simulink model "adc_behavioral"  (R2026a)
settings: Solver=FixedStepDiscrete  StartTime=0  StopTime=4095  FixedStep=1
model workspace (MAT data in the model file):
  C.digital_mode = 3
  C.initial1 = [1 1 1 1]
  C.initial2 = [1 1 1 1]
  C.initial_analog = [0 0 0]
  C.mu1 = [3.81469726563e-09 1.14440917969e-08 2.28881835938e-08 4.57763671875e-08]
  C.mu2 = [6.103515625e-08 1.8310546875e-07 3.662109375e-07 7.32421875e-07]
  C.aux1_gain = 1
  C.aux1_offset = 0
  C.dither_amplitude = 0.03125
  C.copy1 = 64
  C.copy2 = 16
  C.s1_thresholds = [-0.875 -0.625 -0.375 -0.125 0.125 0.375 0.625 0.875]
  C.s1_levels = [-1 -0.75 -0.5 -0.25 0 0.25 0.5 0.75 1]
  C.s1_errors = [0 0 0 0 0 0 0 0 0]
  C.s1_gain = 4
  C.s1_analog = [1 0.975 -0.055 1 0 0.25 0.5 0.75 1 0 0.25 0.5 0.75 1]
  C.s1_phase = [0 0.04 1 0]
  C.s2_thresholds = [-0.875 -0.625 -0.375 -0.125 0.125 0.375 0.625 0.875]
  C.s2_levels = [-1 -0.75 -0.5 -0.25 0 0.25 0.5 0.75 1]
  C.s2_errors = [0 0 0 0 0 0 0 0 0]
  C.s2_gain = 4
  C.s2_analog = [1 0.98 -0.04 1 0 0.25 0.5 0.75 1 0 0.25 0.5 0.75 1]
  C.s2_phase = [0 0.03 1 0]
  C.aux_parameters = [0 1 0 4 4 1 0 1 0.06 1 0]
  d1_signal = [0 1 2 3 4 5 6 7 8 9 10 11 ... (8192 elements, 4096x2)]
  d2_signal = [0 1 2 3 4 5 6 7 8 9 10 11 ... (8192 elements, 4096x2)]
  n_signal = [0 1 2 3 4 5 6 7 8 9 10 11 ... (8192 elements, 4096x2)]
  x_signal = [0 1 2 3 4 5 6 7 8 9 10 11 ... (8192 elements, 4096x2)]
values from neighbouring files (symbols this model uses):
  C = entry.parameters    [adc_load_case.m]    (also in audit_adc_model.m = evalin(workspace,'C'))
(part 1 of 2)
Description:
  | Gu behavioral ADC: independent Simulink implementation, one tick per conversion.
settings Model: Creator=17765  LastModifiedBy=17765

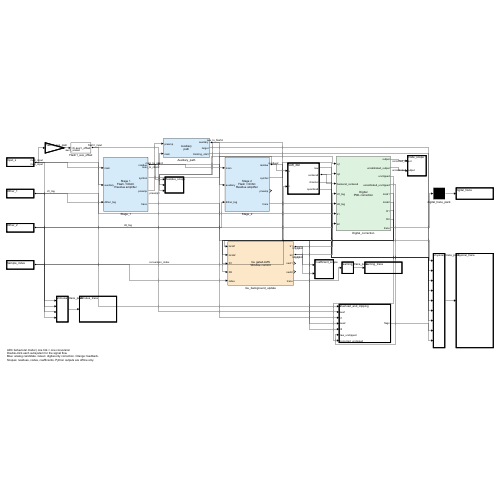
[thumbnail: Simulink's stored preview of the top-level diagram]
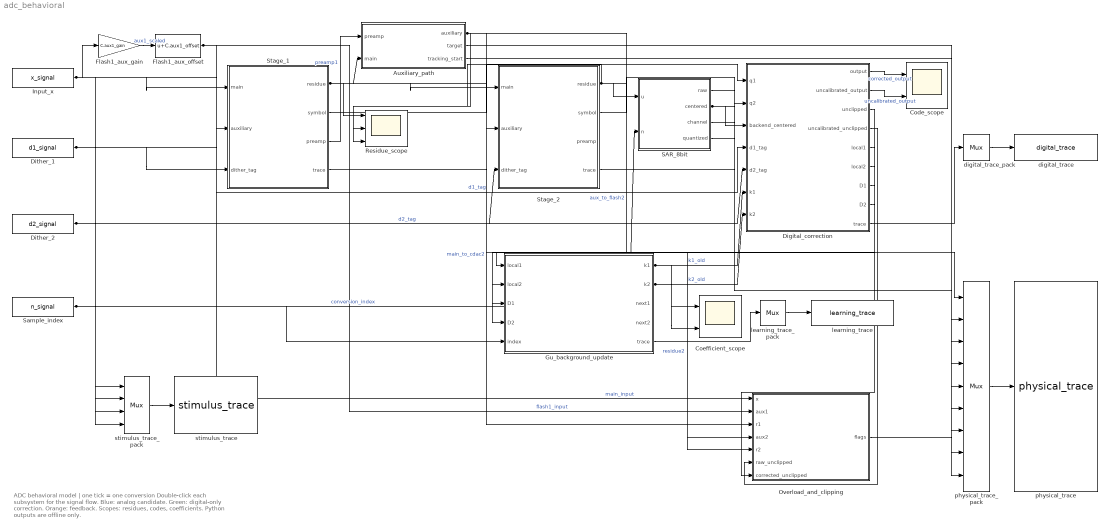
== system adc_behavioral ==
  note: ADC behavioral model | one tick = one conversion
      | Double-click each subsystem for the signal flow.
      | Blue: analog candidate. Green: digital-only correction. Orange: feedback.
      | Scopes: residues, codes, coefficients. Python outputs are offline only.
  Auxiliary_path : Subsystem
      settings: OpenFcn=open_system(gcb,'force')
      mask Display: disp(sprintf('Auxiliary\npath'));
  Code_scope : Scope  NumInputPorts=2
  Coefficient_scope : Scope  NumInputPorts=2
  Digital_correction : Subsystem
      settings: OpenFcn=open_system(gcb,'force')
      mask Display: disp(sprintf('Digital\nPWL correction'));
  Dither_1 : FromWorkspace  VariableName=d1_signal  SampleTime=1  Interpolate=off  OutputAfterFinalValue=Holding final value
  Dither_2 : FromWorkspace  VariableName=d2_signal  SampleTime=1  Interpolate=off  OutputAfterFinalValue=Holding final value
  Flash1_aux_gain : Gain  Gain=C.aux1_gain
  Flash1_aux_offset : Bias  Bias=C.aux1_offset  SaturateOnIntegerOverflow=off
  Gu_background_update : Subsystem
      settings: OpenFcn=open_system(gcb,'force')
      mask Display: disp(sprintf('Gu gated-LMS\nWindow commit'));
  Input_x : FromWorkspace  VariableName=x_signal  SampleTime=1  Interpolate=off  OutputAfterFinalValue=Holding final value
  Overload_and_clipping : MATLAB Function  TreatAsAtomicUnit=on
  Residue_scope : Scope  NumInputPorts=3
  SAR_8bit : MATLAB Function  TreatAsAtomicUnit=on
  Sample_index : FromWorkspace  VariableName=n_signal  SampleTime=1  Interpolate=off  OutputAfterFinalValue=Holding final value
  Stage_1 : Subsystem
      settings: OpenFcn=open_system(gcb,'force')
      mask Display: disp(sprintf('Stage 1\nFlash / CDAC\nResidue amplifier'));
  Stage_2 : Subsystem
      settings: OpenFcn=open_system(gcb,'force')
      mask Display: disp(sprintf('Stage 2\nFlash / CDAC\nResidue amplifier'));
  digital_trace : ToWorkspace  VariableName=digital_trace  SampleTime=1
  digital_trace_pack : Mux  Inputs=1
  learning_trace : ToWorkspace  VariableName=learning_trace  SampleTime=1
  learning_trace_pack : Mux  Inputs=1
  physical_trace : ToWorkspace  VariableName=physical_trace  SampleTime=1
  physical_trace_pack : Mux  Inputs=9
  stimulus_trace : ToWorkspace  VariableName=stimulus_trace  SampleTime=1
  stimulus_trace_pack : Mux
  wires:
  Input_x/1 -> Flash1_aux_gain/1, Stage_1/1(main), Overload_and_clipping/1(x), stimulus_trace_pack/2  "main_input"
  Flash1_aux_gain/1 -> Flash1_aux_offset/1  "aux1_scaled"
  Flash1_aux_offset/1 -> Stage_1/2(auxiliary), Overload_and_clipping/2(aux1)  "flash1_input"
  Dither_1/1 -> Stage_1/3(dither_tag), Digital_correction/4(d1_tag), stimulus_trace_pack/3  "d1_tag"
  Stage_1/3(preamp) -> Auxiliary_path/1(preamp)  "preamp1"
  Stage_1/1(residue) -> Auxiliary_path/2(main), Stage_2/1(main), Residue_scope/1, Overload_and_clipping/3(r1)  "main_to_cdac2"
  Auxiliary_path/1(auxiliary) -> Stage_2/2(auxiliary), Residue_scope/2, Overload_and_clipping/4(aux2)  "aux_to_flash2"
  Dither_2/1 -> Stage_2/3(dither_tag), Digital_correction/5(d2_tag), stimulus_trace_pack/4  "d2_tag"
  Stage_2/1(residue) -> SAR_8bit/1(u), Residue_scope/3, Overload_and_clipping/5(r2)  "residue2"
  Sample_index/1 -> SAR_8bit/2(n), Gu_background_update/5(index), stimulus_trace_pack/1  "conversion_index"
  Stage_1/2(symbol) -> Digital_correction/1(q1)
  Stage_2/2(symbol) -> Digital_correction/2(q2)
  SAR_8bit/2(centered) -> Digital_correction/3(backend_centered), physical_trace_pack/6
  Gu_background_update/1(k1) -> Digital_correction/6(k1), Coefficient_scope/1  "k1_old"
  Gu_background_update/2(k2) -> Digital_correction/7(k2), Coefficient_scope/2  "k2_old"
  Digital_correction/5(local1) -> Gu_background_update/1(local1)
  Digital_correction/6(local2) -> Gu_background_update/2(local2)
  Digital_correction/7(D1) -> Gu_background_update/3(D1)
  Digital_correction/8(D2) -> Gu_background_update/4(D2)
  Digital_correction/1(output) -> Code_scope/1  "corrected_output"
  Digital_correction/2(uncalibrated_output) -> Code_scope/2  "uncalibrated_output"
  Digital_correction/4(uncalibrated_unclipped) -> Overload_and_clipping/6(raw_unclipped)
  Digital_correction/3(unclipped) -> Overload_and_clipping/7(corrected_unclipped)
  Stage_1/4(trace) -> physical_trace_pack/1
  Stage_2/4(trace) -> physical_trace_pack/2
  Auxiliary_path/2(target) -> physical_trace_pack/3
  Auxiliary_path/3(tracking_start) -> physical_trace_pack/4
  SAR_8bit/1(raw) -> physical_trace_pack/5
  SAR_8bit/3(channel) -> physical_trace_pack/7
  SAR_8bit/4(quantized) -> physical_trace_pack/8
  Overload_and_clipping/1(flags) -> physical_trace_pack/9
  physical_trace_pack/1 -> physical_trace/1
  Digital_correction/9(trace) -> digital_trace_pack/1
  digital_trace_pack/1 -> digital_trace/1
  Gu_background_update/5(trace) -> learning_trace_pack/1
  learning_trace_pack/1 -> learning_trace/1
  stimulus_trace_pack/1 -> stimulus_trace/1
